simulink model "sf_execute_at_initialization"  (R2025b)
settings: Solver=FixedStepDiscrete  StartTime=0.0  StopTime=10.0  FixedStep=0.1  RelTol=1e-3  EnableMultiTasking=on
settings Model: Creator=The MathWorks, Inc.  LastModifiedBy=The MathWorks, Inc.
settings SolverCC: AlgebraicLoopSolver=TrustRegion  AutoInsertRateTranBlk=on
settings DataIOCC: LimitDataPoints=on
settings OptimizationCC: LifeSpan=inf
settings DebuggingCC: UnconnectedInputMsg=warning  UnconnectedOutputMsg=warning  UnconnectedLineMsg=warning  AllowSymbolicDim=off  SFUnexpectedBacktrackingDiag=warning  SFNoUnconditionalDefaultTransitionDiag=warning  SFExecutionAtInitializationDiag=none  ArithmeticOperatorsInVariantConditions=warning
settings ModelReferenceCC: EnableRefExpFcnMdlSchedulingChecks=on
settings SFSimCC: SimUseLocalCustomCode=off  CustomCodeUndefinedFunction=UseInterfaceOnly
settings RTWCC: RTWUseLocalCustomCode=off  GPUComputeCapability=3.5  DLArmComputeVersion=19.05
settings CodeAppCC: StateflowObjectComments=on
settings GRTTargetCC: TargetLangStandard=C89/C90 (ANSI)
settings ConfigComp: CovMetricSettings=dw  CovSaveCumulativeToWorkspaceVar=on  CovSaveSingleToWorkspaceVar=on  CovExternalEMLEnable=off

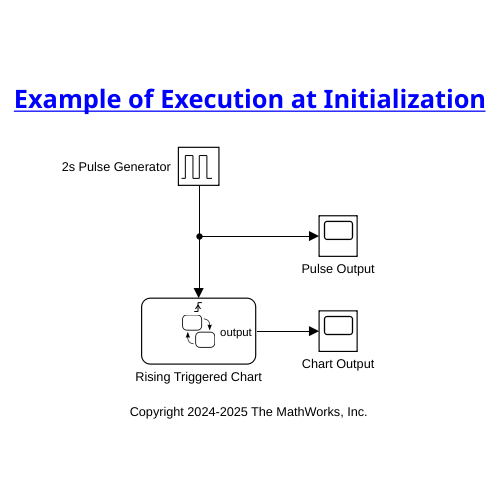
[thumbnail: Simulink's stored preview of the top-level diagram]
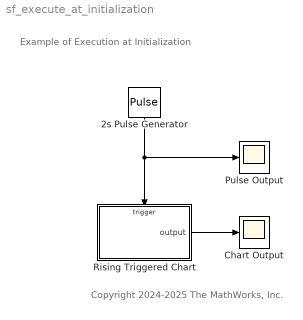
== system sf_execute_at_initialization ==
  note: Copyright 2024-2025 The MathWorks, Inc.
  note: Example of Execution at Initialization
  2s Pulse Generator : DiscretePulseGenerator  PulseType=Time based  PulseWidth=5  PhaseDelay=2
  Chart Output : Scope
      settings: ActiveDisplayYMinimum=0  ActiveDisplayYMaximum=2.125  DataLoggingSaveFormat=Array
  Pulse Output : Scope
      settings: ActiveDisplayYMinimum=-0.125  ActiveDisplayYMaximum=1.125
  Rising Triggered Chart : Stateflow chart  TreatAsAtomicUnit=on
  wires:
  2s Pulse Generator/1 -> Rising Triggered Chart/Trigger, Pulse Output/1
  Rising Triggered Chart/1(output) -> Chart Output/1

== stateflow chart sf_execute_at_initialization/Rising Triggered Chart ==
  settings: executeAtInitialization=1
  state Set_Output
    entry: output = 1;
    during: output = 2;
  (default) -> Set_Output
  data: output output =0
  events: event input RISING_EDGE_EVENT
